simulink model "s_c_nbe_m32k"  (R2018a)
settings: Solver=VariableStepDiscrete  StartTime=0.0  StopTime=1000  RelTol=1e-3
undefined symbols (not defined in the file): fft_stages, n_taps, output_bits, pfb_coeff_gen_calc, xengbits
libraries: xbsIndex_r4 x23714, casper_library_misc x17, xps_library x4, casper_library_scopes x4, xbsReplacements_r4 x4
(part 18 of 171)

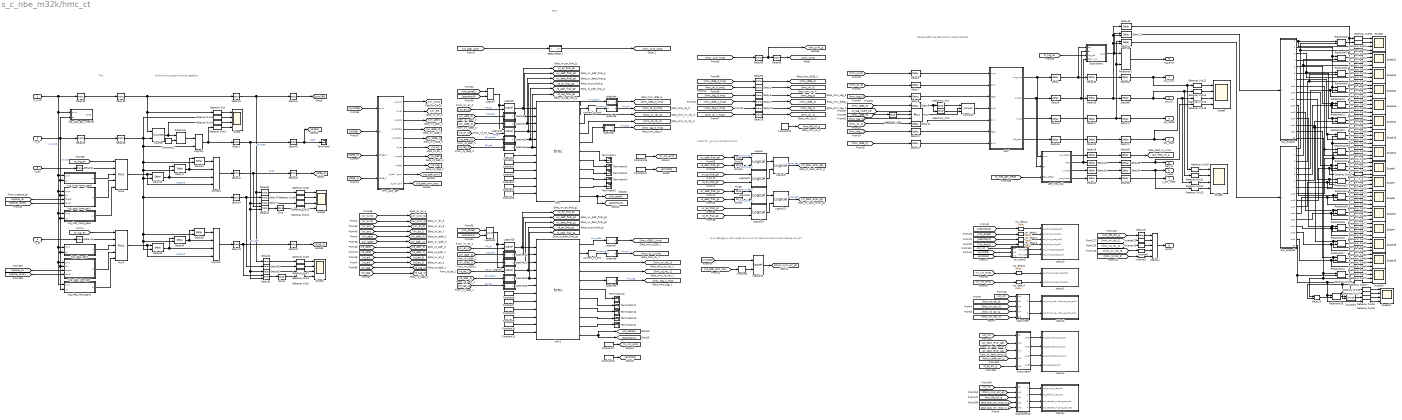
== system s_c_nbe_m32k/hmc_ct ==
  note: Double buffer the data to form output packets
  note: TVG
  note: Write two successive words together.
  note: Sync debugging - did we get two syncs
      | so close we weren't even reading out yet?
  note: Check for _en sync and bank errors
  note: HMC
  in_sync : Inport
  in_dv : Inport  Port=2
  in_d0 : Inport  Port=3
  in_d1 : Inport  Port=4
  Concat13 : xbsIndex_r4/Concat  num_inputs=3  dbl_ovrd=off  block_type=concat
  Concat2 : xbsIndex_r4/Concat  num_inputs=4  dbl_ovrd=off  block_type=concat
  Concat3 : xbsIndex_r4/Concat  num_inputs=4  dbl_ovrd=off  block_type=concat
  Constant{,3,6,9} (4 alike) : xbsIndex_r4/Constant  const=0  gui_display_data_type=Boolean  arith_type=Boolean  n_bits=16  bin_pt=14  preci_type=Single  exp_width=8  frac_width=24  explicit_period=on  period=1  equ=P=C  opselect=C  inp2=PCIN>>17  opr=+  inp1=P  carry=CIN  dbl_ovrd=off  block_type=constant
  Constant{1,4,7,10} (4 alike) : xbsIndex_r4/Constant  const=0  gui_display_data_type=Fixed-point  arith_type=Unsigned  n_bits=27  bin_pt=0  preci_type=Single  exp_width=8  frac_width=24  explicit_period=on  period=1  equ=P=C  opselect=C  inp2=PCIN>>17  opr=+  inp1=P  carry=CIN  dbl_ovrd=off  block_type=constant
  Constant11 : xbsIndex_r4/Constant  const=0  gui_display_data_type=Fixed-point  arith_type=Unsigned  n_bits=9  bin_pt=0  preci_type=Single  exp_width=8  frac_width=24  explicit_period=on  period=1  equ=P=C  opselect=C  inp2=PCIN>>17  opr=+  inp1=P  carry=CIN  dbl_ovrd=off  block_type=constant
  Constant12 : xbsIndex_r4/Constant  const=3  gui_display_data_type=Fixed-point  arith_type=Unsigned  n_bits=2  bin_pt=0  preci_type=Single  exp_width=8  frac_width=24  explicit_period=on  period=1  equ=P=C  opselect=C  inp2=PCIN>>17  opr=+  inp1=P  carry=CIN  dbl_ovrd=off  block_type=constant
  Constant13 : xbsIndex_r4/Constant  const=0  gui_display_data_type=Boolean  arith_type=Boolean  n_bits=1  bin_pt=0  preci_type=Single  exp_width=8  frac_width=24  explicit_period=on  period=1  equ=P=C  opselect=C  inp2=PCIN>>17  opr=+  inp1=P  carry=CIN  dbl_ovrd=off  block_type=constant
  Constant14 : xbsIndex_r4/Constant  const=0  gui_display_data_type=Fixed-point  arith_type=Unsigned  n_bits=7  bin_pt=0  preci_type=Single  exp_width=8  frac_width=24  explicit_period=on  period=1  equ=P=C  opselect=C  inp2=PCIN>>17  opr=+  inp1=P  carry=CIN  dbl_ovrd=off  block_type=constant
  Constant15 : xbsIndex_r4/Constant  const=0  gui_display_data_type=Fixed-point  arith_type=Unsigned  n_bits=16  bin_pt=0  preci_type=Single  exp_width=8  frac_width=24  explicit_period=on  period=1  equ=P=C  opselect=C  inp2=PCIN>>17  opr=+  inp1=P  carry=CIN  dbl_ovrd=off  block_type=constant
  Constant16 : xbsIndex_r4/Constant  const=0  gui_display_data_type=Fixed-point  arith_type=Unsigned  n_bits=7  bin_pt=0  preci_type=Single  exp_width=8  frac_width=24  explicit_period=on  period=1  equ=P=C  opselect=C  inp2=PCIN>>17  opr=+  inp1=P  carry=CIN  dbl_ovrd=off  block_type=constant
  Constant17 : xbsIndex_r4/Constant  const=0  gui_display_data_type=Fixed-point  arith_type=Unsigned  n_bits=16  bin_pt=0  preci_type=Single  exp_width=8  frac_width=24  explicit_period=on  period=1  equ=P=C  opselect=C  inp2=PCIN>>17  opr=+  inp1=P  carry=CIN  dbl_ovrd=off  block_type=constant
  Constant2 : xbsIndex_r4/Constant  const=0  gui_display_data_type=Fixed-point  arith_type=Unsigned  n_bits=256  bin_pt=0  preci_type=Single  exp_width=8  frac_width=24  explicit_period=on  period=1  equ=P=C  opselect=C  inp2=PCIN>>17  opr=+  inp1=P  carry=CIN  dbl_ovrd=off  block_type=constant
  Constant5 : xbsIndex_r4/Constant  const=0  gui_display_data_type=Fixed-point  arith_type=Unsigned  n_bits=9  bin_pt=0  preci_type=Single  exp_width=8  frac_width=24  explicit_period=on  period=1  equ=P=C  opselect=C  inp2=PCIN>>17  opr=+  inp1=P  carry=CIN  dbl_ovrd=off  block_type=constant
  Constant8 : xbsIndex_r4/Constant  const=0  gui_display_data_type=Fixed-point  arith_type=Unsigned  n_bits=256  bin_pt=0  preci_type=Single  exp_width=8  frac_width=24  explicit_period=on  period=1  equ=P=C  opselect=C  inp2=PCIN>>17  opr=+  inp1=P  carry=CIN  dbl_ovrd=off  block_type=constant
  Counter : xbsIndex_r4/Counter  cnt_type=Free Running  cnt_to=Inf  operation=Up  start_count=0  cnt_by_val=1  arith_type=Unsigned  n_bits=2  bin_pt=0  load_pin=off  rst=on  en=on  explicit_period=on  period=1  use_behavioral_HDL=off  implementation=Fabric  dbl_ovrd=off  block_type=counter
  Counter1 : xbsIndex_r4/Counter  cnt_type=Free Running  cnt_to=Inf  operation=Up  start_count=0  cnt_by_val=1  arith_type=Unsigned  n_bits=8  bin_pt=0  load_pin=off  rst=on  en=on  explicit_period=on  period=1  use_behavioral_HDL=off  implementation=Fabric  dbl_ovrd=off  block_type=counter
  Delay{,6,10,16} (4 alike) : xbsIndex_r4/Delay  rst=off  infoeditControl=Selection of Reset will increase slice count due to use of real FFs and instead of SRLs  en=off  latency=21  reg_retiming=on  dbl_ovrd=off  block_type=delay
      settings: infoedit=Hardware notes: A delay line is a chain, each link of which is an SRL16 or SRL32 followed by a flip-flop.
  Delay{1,5,7..9,11..13,15,25..29,35,39..40,42,54,61..62,78,93} (23 alike) : xbsIndex_r4/Delay  rst=off  infoeditControl=Selection of Reset will increase slice count due to use of real FFs and instead of SRLs  en=off  latency=2  reg_retiming=on  dbl_ovrd=off  block_type=delay
      settings: infoedit=Hardware notes: A delay line is a chain, each link of which is an SRL16 or SRL32 followed by a flip-flop.
  Delay{14,21..23,81} (5 alike) : xbsIndex_r4/Delay  rst=off  infoeditControl=Selection of Reset will increase slice count due to use of real FFs and instead of SRLs  en=on  latency=1  reg_retiming=off  dbl_ovrd=off  block_type=delay
      settings: infoedit=Hardware notes: A delay line is a chain, each link of which is an SRL16 or SRL32 followed by a flip-flop.
  Delay{2..4,17..19,43..45,63,66,72..73,75,85..86,89..90,94..95} (20 alike) : xbsIndex_r4/Delay  rst=off  infoeditControl=Selection of Reset will increase slice count due to use of real FFs and instead of SRLs  en=off  latency=1  reg_retiming=on  dbl_ovrd=off  block_type=delay
      settings: infoedit=Hardware notes: A delay line is a chain, each link of which is an SRL16 or SRL32 followed by a flip-flop.
  Delay{33..34,36,41} (4 alike) : xbsIndex_r4/Delay  rst=off  infoeditControl=Selection of Reset will increase slice count due to use of real FFs and instead of SRLs  en=off  latency=4  reg_retiming=on  dbl_ovrd=off  block_type=delay
      settings: infoedit=Hardware notes: A delay line is a chain, each link of which is an SRL16 or SRL32 followed by a flip-flop.
  Delay{46..47,51,60,64..65} (6 alike) : xbsIndex_r4/Delay  rst=off  infoeditControl=Selection of Reset will increase slice count due to use of real FFs and instead of SRLs  en=on  latency=1  reg_retiming=on  dbl_ovrd=off  block_type=delay
      settings: infoedit=Hardware notes: A delay line is a chain, each link of which is an SRL16 or SRL32 followed by a flip-flop.
  Delay{48,77,79..80,82..84} (7 alike) : xbsIndex_r4/Delay  rst=off  infoeditControl=Selection of Reset will increase slice count due to use of real FFs and instead of SRLs  en=off  latency=1  reg_retiming=off  dbl_ovrd=off  block_type=delay
      settings: infoedit=Hardware notes: A delay line is a chain, each link of which is an SRL16 or SRL32 followed by a flip-flop.
  Gateway Out{,1..87} (88 alike) : xbsIndex_r4/Gateway Out  inherit_from_input=off  hdl_port=off  rows=1  columns=1  UseAsDAC=off  DACChannel='1'  interface=None  automatic_assignment=on  address_offset=hex2dec('00')  intf_name=''  intf_description=''  timing_constraint=None  locs_specified=off  LOCs={}  io_standard={}  block_type=gatewayout
  Inverter{1..2,22..23} (4 alike) : xbsIndex_r4/Inverter  en=off  latency=1  dbl_ovrd=off  block_type=inv
  Inverter6 : xbsIndex_r4/Inverter  en=off  latency=0  dbl_ovrd=off  block_type=inv
  Logical{,1,8,19,21} (5 alike) : xbsIndex_r4/Logical  logical_function=AND  inputs=2  en=off  latency=0  precision=Full  arith_type=Unsigned  n_bits=16  bin_pt=0  align_bp=on  dbl_ovrd=off  block_type=logical
  Logical10 : xbsIndex_r4/Logical  logical_function=OR  inputs=2  en=off  latency=0  precision=Full  arith_type=Unsigned  n_bits=16  bin_pt=0  align_bp=on  dbl_ovrd=off  block_type=logical
  Logical{2,5,11,15,18} (5 alike) : xbsIndex_r4/Logical  logical_function=AND  inputs=2  en=off  latency=2  precision=Full  arith_type=Unsigned  n_bits=16  bin_pt=0  align_bp=on  dbl_ovrd=off  block_type=logical
  Logical20 : xbsIndex_r4/Logical  logical_function=OR  inputs=2  en=off  latency=0  precision=Full  arith_type=Unsigned  n_bits=16  bin_pt=0  align_bp=on  dbl_ovrd=off  block_type=logical
  Logical28 : xbsIndex_r4/Logical  logical_function=AND  inputs=2  en=off  latency=1  precision=Full  arith_type=Unsigned  n_bits=16  bin_pt=0  align_bp=on  dbl_ovrd=off  block_type=logical
  Logical4 : xbsIndex_r4/Logical  logical_function=OR  inputs=5  en=off  latency=1  precision=Full  arith_type=Unsigned  n_bits=16  bin_pt=0  align_bp=on  dbl_ovrd=off  block_type=logical
  Logical7 : xbsIndex_r4/Logical  logical_function=AND  inputs=2  en=off  latency=1  precision=Full  arith_type=Unsigned  n_bits=16  bin_pt=0  align_bp=on  dbl_ovrd=off  block_type=logical
  Mux : xbsIndex_r4/Mux  inputs=2  en=off  latency=2  precision=Full  arith_type=Unsigned  n_bits=16  bin_pt=14  quantization=Truncate  overflow=Wrap  dbl_ovrd=off  block_type=mux
  Mux3 : xbsIndex_r4/Mux  inputs=4  en=off  latency=2  precision=Full  arith_type=Unsigned  n_bits=16  bin_pt=14  quantization=Truncate  overflow=Wrap  dbl_ovrd=off  block_type=mux
  Mux4 : xbsIndex_r4/Mux  inputs=4  en=off  latency=2  precision=Full  arith_type=Unsigned  n_bits=16  bin_pt=14  quantization=Truncate  overflow=Wrap  dbl_ovrd=off  block_type=mux
  Relational : xbsIndex_r4/Relational  mode=a=b  op_type=Bool  en=off  latency=0  dbl_ovrd=off  block_type=relational
  Relational1 : xbsIndex_r4/Relational  mode=a!=b  op_type=Bool  en=off  latency=1  dbl_ovrd=off  block_type=relational
  Relational{2..18} (17 alike) : xbsIndex_r4/Relational  mode=a!=b  op_type=Bool  en=off  latency=0  dbl_ovrd=off  block_type=relational
  Scope{,1..21} (22 alike) : Scope  NumInputPorts=4
  Slice : xbsIndex_r4/Slice  nbits=16  boolean_output=off  mode=Upper Bit Location + Width  bit1=0  base1=MSB of Input  bit0=0  base0=LSB of Input  dbl_ovrd=off  block_type=slice
  Slice1 : xbsIndex_r4/Slice  nbits=16  boolean_output=off  mode=Upper Bit Location + Width  bit1=0  base1=MSB of Input  bit0=0  base0=LSB of Input  dbl_ovrd=off  block_type=slice
  Slice{8..9,12..13} (4 alike) : xbsIndex_r4/Slice  nbits=1  boolean_output=on  mode=Lower Bit Location + Width  bit1=0  base1=MSB of Input  bit0=input_len_bits - 2 + output_len_bits  base0=LSB of Input  dbl_ovrd=off  block_type=slice
  Subsystem : Subsystem
  Subsystem1 : Subsystem
  Subsystem22 : Subsystem  mask{n_bits_count=8}
      mask prompts: n_bits_count "Counter bits"
  Subsystem9 : Subsystem  mask{n_bits_count=8}
      mask prompts: n_bits_count "Counter bits"
  Terminator{,1..5,10..14} (11 alike) : Terminator
  bus_expand : Subsystem  mask(bus_expand){mode=divisions of equal size, outputNum=16, outputWidth=16, outputBinaryPt=0, outputArithmeticType=0, show_format=off, outputToWorkspace=off, variablePrefix=out, outputToModelAsWell=on}
      mask prompts: outputNum "Number of outputs:"; outputWidth "Output width:"; outputBinaryPt "Output binary point position:"; outputArithmeticType "Output arithmetic type (ufix=0, fix=1, bool=2):"; show_format "Print format string?"; outputToWorkspace "Output to workspace?"; variablePrefix "Variable name prefix:"; outputToModelAsWell "Output to model as well?"
      mask help:
      | Expands a 'bus' made using a bus_create or Xilinx
      | concat block.
      | The input will be divided into the specified number
      | of outputs with the specified arithmetic types.
      | Divisions are made from most significant bit.
      mask init: same as s_c_nbe_m32k/bus_expand1
      settings: AttributesFormatString=16 outputs
      mask TypeOptions mode: divisions of equal size | divisions of arbitrary size
      mask Callback mode: bus_expand_callback();
      mask Callback outputWidth: bus_expand_callback();
      mask Callback outputToWorkspace: bus_expand_callback();
  bus_expand1 : Subsystem  mask(bus_expand){mode=divisions of equal size, outputNum=16, outputWidth=16, outputBinaryPt=0, outputArithmeticType=0, show_format=off, outputToWorkspace=off, variablePrefix=out, outputToModelAsWell=on}
      mask prompts: outputNum "Number of outputs:"; outputWidth "Output width:"; outputBinaryPt "Output binary point position:"; outputArithmeticType "Output arithmetic type (ufix=0, fix=1, bool=2):"; show_format "Print format string?"; outputToWorkspace "Output to workspace?"; variablePrefix "Variable name prefix:"; outputToModelAsWell "Output to model as well?"
      mask help:
      | Expands a 'bus' made using a bus_create or Xilinx
      | concat block.
      | The input will be divided into the specified number
      | of outputs with the specified arithmetic types.
      | Divisions are made from most significant bit.
      mask init: same as s_c_nbe_m32k/bus_expand1
      settings: AttributesFormatString=16 outputs
      mask TypeOptions mode: divisions of equal size | divisions of arbitrary size
      mask Callback mode: bus_expand_callback();
      mask Callback outputWidth: bus_expand_callback();
      mask Callback outputToWorkspace: bus_expand_callback();
  convert_rd_en1 : xbsIndex_r4/Convert  gui_display_data_type=Boolean  arith_type=Boolean  n_bits=128  bin_pt=0  float_type=Single  exp_bits=8  fraction_bits=24  quantization=Truncate  overflow=Wrap  en=off  latency=0  pipeline=off  dbl_ovrd=off  block_type=convert
      settings: xl_area=[0, 0, 0, 0, 0, 0, 0]
  convert_rd_en4 : xbsIndex_r4/Convert  gui_display_data_type=Boolean  arith_type=Boolean  n_bits=128  bin_pt=0  float_type=Single  exp_bits=8  fraction_bits=24  quantization=Truncate  overflow=Wrap  en=off  latency=0  pipeline=off  dbl_ovrd=off  block_type=convert
      settings: xl_area=[0, 0, 0, 0, 0, 0, 0]
  edge_detect1 : Subsystem  mask(edge_detect){edge=Rising, polarity=Active High, x_in=[0 0.08 0.08 0.16 0.16 0.24 0.24 0.32 0.32 0.4], y_in=[-1 -1  1  1  1  1  1  1  1  1], x_out=[0.6 0.68 0.68 0.76 0.76 0.84 0.84 0.92 0.92 1], y_out=[-1 -1  1  1 -1 -1 -1 -1 -1 -1]}
      mask prompts: edge "Edge Type"; polarity "Output Polarity"; x_in "Input X Positions"; y_in "Input Y Positions"; x_out "Output X Positions"; y_out "Output Y Positions"
      mask help: Output is active for one-cycle after each edge of the specified type (i.e. rising, falling or both).
      mask init: same as s_c_nbe_m32k/edge_detect1
      settings: AttributesFormatString=|
      | rising edges
      | active high
      mask Help: Output is active for one-cycle after each edge of the specified type (i.e. rising, falling, or both).  Latency is zero.
      mask TypeOptions edge: Rising | Falling | Both
      mask TypeOptions polarity: Active High | Active Low
      mask Display:
      | plot(x_in_num,0.5+y_in_num*0.2);
      | plot(x_out_num,0.5+y_out_num*0.2);
  err_latch3 : Subsystem
  gen_freq_calc : Subsystem  mask{pkt_len_bits=5, lat=3}
      mask prompts: pkt_len_bits "Packet length bits"; lat "Latency"
      mask init:
      | display_string = sprintf('latency=%i', 7 * lat);
      | set_param(gcb, 'AttributesFormatString', display_string);
      settings: AttributesFormatString=latency=21
  hmc : xps_library/Memory/hmc  Tag=xps:hmc  mez=1  sim_depth=(input_len_bits-1) + output_len_bits + 1  sim_latency=5  sim_rand=on
      settings: SourceProductName=CASPER XPS Blockset
  hmc1 : xps_library/Memory/hmc  Tag=xps:hmc  mez=2  sim_depth=(input_len_bits-1) + output_len_bits + 1  sim_latency=5  sim_rand=on
      settings: SourceProductName=CASPER XPS Blockset
  hmc_addr_gen : Subsystem  mask{invec_bits=input_len_bits-2, outvec_bits=output_len_bits, max_x_boards_bits=max_x_boards_bits, max_x_per_board_bits=max_x_per_board_bits, n_bits_chans_per_word=4}
      mask prompts: invec_bits "Input vector bits"; outvec_bits "Output vector bits"; max_x_boards_bits "Max number x boards (2^?)"; max_x_per_board_bits "max xengines per board (2^?)"; n_bits_chans_per_word "channels per input word (2^?)"
      mask init:
      | vec_len = 2^invec_bits * 2^outvec_bits;
      | mystr = sprintf('2^%i x 2^%i = %i', invec_bits, outvec_bits, vec_len);
      | set_param(gcb, 'AttributesFormatString', mystr);
      settings: AttributesFormatString=2^11 x 2^8 = 524288
  obuf : Subsystem  mask{output_vec_bits=output_len_bits, pkt_buffer_latency=4, omux_latency=3}
      mask prompts: output_vec_bits "CT output vector bits"; pkt_buffer_latency "Output buffer latency"; omux_latency "Output mux latency"
  pipeline : Subsystem  Tag=cmac_delinked  mask(pipeline){csp_latency=2}
      mask prompts: csp_latency "Latency"
      mask help:
      | An explicitly laid-out delay line to avoid mapping to SRL16s
      | for use in pipelining to help achieve timing closure.
      mask init:
      | pipeline_init(gcb,'latency',csp_latency);
      settings: AttributesFormatString=Latency = %<latency>
      mask Display:
      | port_label('input', 1, 'd');
      | port_label('output', 1, 'q');
      | disp(['Z^-', num2str(csp_latency)]);
  pipeline1 : Subsystem  Tag=cmac_delinked  mask(pipeline){csp_latency=2}
      mask prompts: csp_latency "Latency"
      mask help:
      | An explicitly laid-out delay line to avoid mapping to SRL16s
      | for use in pipelining to help achieve timing closure.
      mask init:
      | pipeline_init(gcb,'latency',csp_latency);
      settings: AttributesFormatString=Latency = %<latency>
      mask Display:
      | port_label('input', 1, 'd');
      | port_label('output', 1, 'q');
      | disp(['Z^-', num2str(csp_latency)]);
  pipeline10 : Subsystem  Tag=cmac_delinked  mask(pipeline){csp_latency=2}
      mask prompts: csp_latency "Latency"
      mask help:
      | An explicitly laid-out delay line to avoid mapping to SRL16s
      | for use in pipelining to help achieve timing closure.
      mask init:
      | pipeline_init(gcb,'latency',csp_latency);
      settings: AttributesFormatString=Latency = %<latency>
      mask Display:
      | port_label('input', 1, 'd');
      | port_label('output', 1, 'q');
      | disp(['Z^-', num2str(csp_latency)]);
  pipeline11 : Subsystem  Tag=cmac_delinked  mask(pipeline){csp_latency=2}
      mask prompts: csp_latency "Latency"
      mask help:
      | An explicitly laid-out delay line to avoid mapping to SRL16s
      | for use in pipelining to help achieve timing closure.
      mask init:
      | pipeline_init(gcb,'latency',csp_latency);
      settings: AttributesFormatString=Latency = %<latency>
      mask Display:
      | port_label('input', 1, 'd');
      | port_label('output', 1, 'q');
      | disp(['Z^-', num2str(csp_latency)]);
  pipeline12 : Subsystem  Tag=cmac_delinked  mask(pipeline){csp_latency=2}
      mask prompts: csp_latency "Latency"
      mask help:
      | An explicitly laid-out delay line to avoid mapping to SRL16s
      | for use in pipelining to help achieve timing closure.
      mask init:
      | pipeline_init(gcb,'latency',csp_latency);
      settings: AttributesFormatString=Latency = %<latency>
      mask Display:
      | port_label('input', 1, 'd');
      | port_label('output', 1, 'q');
      | disp(['Z^-', num2str(csp_latency)]);
  pipeline13 : Subsystem  Tag=cmac_delinked  mask(pipeline){csp_latency=2}
      mask prompts: csp_latency "Latency"
      mask help:
      | An explicitly laid-out delay line to avoid mapping to SRL16s
      | for use in pipelining to help achieve timing closure.
      mask init:
      | pipeline_init(gcb,'latency',csp_latency);
      settings: AttributesFormatString=Latency = %<latency>
      mask Display:
      | port_label('input', 1, 'd');
      | port_label('output', 1, 'q');
      | disp(['Z^-', num2str(csp_latency)]);
  pipeline2 : Subsystem  Tag=cmac_delinked  mask(pipeline){csp_latency=2}
      mask prompts: csp_latency "Latency"
      mask help:
      | An explicitly laid-out delay line to avoid mapping to SRL16s
      | for use in pipelining to help achieve timing closure.
      mask init:
      | pipeline_init(gcb,'latency',csp_latency);
      settings: AttributesFormatString=Latency = %<latency>
      mask Display:
      | port_label('input', 1, 'd');
      | port_label('output', 1, 'q');
      | disp(['Z^-', num2str(csp_latency)]);
  pipeline3 : Subsystem  Tag=cmac_delinked  mask(pipeline){csp_latency=2}
      mask prompts: csp_latency "Latency"
      mask help:
      | An explicitly laid-out delay line to avoid mapping to SRL16s
      | for use in pipelining to help achieve timing closure.
      mask init:
      | pipeline_init(gcb,'latency',csp_latency);
      settings: AttributesFormatString=Latency = %<latency>
      mask Display:
      | port_label('input', 1, 'd');
      | port_label('output', 1, 'q');
      | disp(['Z^-', num2str(csp_latency)]);
  pipeline4 : Subsystem  Tag=cmac_delinked  mask(pipeline){csp_latency=2}
      mask prompts: csp_latency "Latency"
      mask help:
      | An explicitly laid-out delay line to avoid mapping to SRL16s
      | for use in pipelining to help achieve timing closure.
      mask init:
      | pipeline_init(gcb,'latency',csp_latency);
      settings: AttributesFormatString=Latency = %<latency>
      mask Display:
      | port_label('input', 1, 'd');
      | port_label('output', 1, 'q');
      | disp(['Z^-', num2str(csp_latency)]);
  pipeline5 : Subsystem  Tag=cmac_delinked  mask(pipeline){csp_latency=2}
      mask prompts: csp_latency "Latency"
      mask help:
      | An explicitly laid-out delay line to avoid mapping to SRL16s
      | for use in pipelining to help achieve timing closure.
      mask init:
      | pipeline_init(gcb,'latency',csp_latency);
      settings: AttributesFormatString=Latency = %<latency>
      mask Display:
      | port_label('input', 1, 'd');
      | port_label('output', 1, 'q');
      | disp(['Z^-', num2str(csp_latency)]);
  pipeline6 : Subsystem  Tag=cmac_delinked  mask(pipeline){csp_latency=2}
      mask prompts: csp_latency "Latency"
      mask help:
      | An explicitly laid-out delay line to avoid mapping to SRL16s
      | for use in pipelining to help achieve timing closure.
      mask init:
      | pipeline_init(gcb,'latency',csp_latency);
      settings: AttributesFormatString=Latency = %<latency>
      mask Display:
      | port_label('input', 1, 'd');
      | port_label('output', 1, 'q');
      | disp(['Z^-', num2str(csp_latency)]);
  pipeline7 : Subsystem  Tag=cmac_delinked  mask(pipeline){csp_latency=2}
      mask prompts: csp_latency "Latency"
      mask help:
      | An explicitly laid-out delay line to avoid mapping to SRL16s
      | for use in pipelining to help achieve timing closure.
      mask init:
      | pipeline_init(gcb,'latency',csp_latency);
      settings: AttributesFormatString=Latency = %<latency>
      mask Display:
      | port_label('input', 1, 'd');
      | port_label('output', 1, 'q');
      | disp(['Z^-', num2str(csp_latency)]);
  pipeline8 : Subsystem  Tag=cmac_delinked  mask(pipeline){csp_latency=2}
      mask prompts: csp_latency "Latency"
      mask help:
      | An explicitly laid-out delay line to avoid mapping to SRL16s
      | for use in pipelining to help achieve timing closure.
      mask init:
      | pipeline_init(gcb,'latency',csp_latency);
      settings: AttributesFormatString=Latency = %<latency>
      mask Display:
      | port_label('input', 1, 'd');
      | port_label('output', 1, 'q');
      | disp(['Z^-', num2str(csp_latency)]);
  pipeline9 : Subsystem  Tag=cmac_delinked  mask(pipeline){csp_latency=2}
      mask prompts: csp_latency "Latency"
      mask help:
      | An explicitly laid-out delay line to avoid mapping to SRL16s
      | for use in pipelining to help achieve timing closure.
      mask init:
      | pipeline_init(gcb,'latency',csp_latency);
      settings: AttributesFormatString=Latency = %<latency>
      mask Display:
      | port_label('input', 1, 'd');
      | port_label('output', 1, 'q');
      | disp(['Z^-', num2str(csp_latency)]);
  rst_delay{1..5,7} (6 alike) : xbsIndex_r4/Delay  rst=off  infoeditControl=Selection of Reset will increase slice count due to use of real FFs and instead of SRLs  en=off  latency=1  reg_retiming=on  dbl_ovrd=off  block_type=delay
      settings: infoedit=Hardware notes: A delay line is a chain, each link of which is an SRL16 or SRL32 followed by a flip-flop.
  spectrum_ctr2 : xbsIndex_r4/Slice  nbits=256 - (32 + 10)  boolean_output=off  mode=Lower Bit Location + Width  bit1=-1  base1=MSB of Input  bit0=32 + 10  base0=LSB of Input  dbl_ovrd=off  block_type=slice
  spectrum_ctr3 : xbsIndex_r4/Slice  nbits=32  boolean_output=off  mode=Lower Bit Location + Width  bit1=-1  base1=MSB of Input  bit0=0  base0=LSB of Input  dbl_ovrd=off  block_type=slice
  spectrum_ctr4 : xbsIndex_r4/Slice  nbits=10  boolean_output=off  mode=Lower Bit Location + Width  bit1=-1  base1=MSB of Input  bit0=32  base0=LSB of Input  dbl_ovrd=off  block_type=slice
  status0 : Subsystem  Tag=xps:sw_reg  AncestorBlock=xps_library/Memory/software_register  mask(swreg){io_dir=To Processor, io_delay=0, init_val=0, sample_period=1, names=[hmc_post_pol0 hmc_init_pol0 hmc_post_pol1 hmc_init_pol1 hmc_errstat_pol0 hmc_errstat_pol1], bitwidths=[1 1 1 1 7 7], bin_pts=0, arith_types=[2 2 2 2 0 0], sim_port=off, show_format=on}
      mask prompts: io_dir "I/O direction"; io_delay "I/O delay"; init_val "Initial Value"; sample_period "Sample period"; names "Bitfield names [msb...lsb]"; bitwidths "Bitfield widths"; bin_pts "Bitfield binary pts"; arith_types "Bitfield types, ufix=0, fix=1, bool=2"; sim_port "Provide sim input/output?"; show_format "Print format string?"
      mask help: A 32-bit software-accessible register. Can be divided into bitfields of varying widths and types using the fields in the block mask.
      mask init:
      | swreg_init(gcb)
      settings: AttributesFormatString=6 outputs:b,b,b,b,uf7.0,uf7.0 = 18 bits
      mask TypeOptions io_dir: To Processor | From Processor
      mask Callback io_dir:
      | mask_enables = get_param(gcb, 'MaskEnables');
      | mask_names = get_param(gcb, 'MaskNames');
      | if strcmp(get_param(gcb, 'io_dir'), 'To Processor'),
      |     mask_enables{ismember(mask_names, 'sample_period')} = 'off';
      | else
      |     mask_enables{ismember(mask_names, 'sample_period')} = 'on';
      | end
      | set_param(gcb, 'MaskEnables', mask_enables);
      mask DialogControl ParameterTabVar0 Prompt: Setup
  status1 : Subsystem  Tag=xps:sw_reg  AncestorBlock=xps_library/Memory/software_register  mask(swreg){io_dir=To Processor, io_delay=0, init_val=0, sample_period=1, names=[hmc_crc_err_cnt_pol0 hmc_crc_err_cnt_pol1], bitwidths=16, bin_pts=0, arith_types=0, sim_port=off, show_format=on}
      mask prompts: io_dir "I/O direction"; io_delay "I/O delay"; init_val "Initial Value"; sample_period "Sample period"; names "Bitfield names [msb...lsb]"; bitwidths "Bitfield widths"; bin_pts "Bitfield binary pts"; arith_types "Bitfield types, ufix=0, fix=1, bool=2"; sim_port "Provide sim input/output?"; show_format "Print format string?"
      mask help: A 32-bit software-accessible register. Can be divided into bitfields of varying widths and types using the fields in the block mask.
      mask init:
      | swreg_init(gcb)
      settings: AttributesFormatString=2 outputs:uf16.0,uf16.0 = 32 bits
      mask TypeOptions io_dir: To Processor | From Processor
      mask Callback io_dir:
      | mask_enables = get_param(gcb, 'MaskEnables');
      | mask_names = get_param(gcb, 'MaskNames');
      | if strcmp(get_param(gcb, 'io_dir'), 'To Processor'),
      |     mask_enables{ismember(mask_names, 'sample_period')} = 'off';
      | else
      |     mask_enables{ismember(mask_names, 'sample_period')} = 'on';
      | end
      | set_param(gcb, 'MaskEnables', mask_enables);
      mask DialogControl ParameterTabVar0 Prompt: Setup
  status2 : Subsystem  Tag=xps:sw_reg  AncestorBlock=xps_library/Memory/software_register  mask(swreg){io_dir=To Processor, io_delay=0, init_val=0, sample_period=1, names=[hmc_overflow_err_cnt_pol0 hmc_overflow_err_cnt_pol1], bitwidths=16, bin_pts=0, arith_types=0, sim_port=off, show_format=on}
      mask prompts: io_dir "I/O direction"; io_delay "I/O delay"; init_val "Initial Value"; sample_period "Sample period"; names "Bitfield names [msb...lsb]"; bitwidths "Bitfield widths"; bin_pts "Bitfield binary pts"; arith_types "Bitfield types, ufix=0, fix=1, bool=2"; sim_port "Provide sim input/output?"; show_format "Print format string?"
      mask help: A 32-bit software-accessible register. Can be divided into bitfields of varying widths and types using the fields in the block mask.
      mask init:
      | swreg_init(gcb)
      settings: AttributesFormatString=2 outputs:uf16.0,uf16.0 = 32 bits
      mask TypeOptions io_dir: To Processor | From Processor
      mask Callback io_dir:
      | mask_enables = get_param(gcb, 'MaskEnables');
      | mask_names = get_param(gcb, 'MaskNames');
      | if strcmp(get_param(gcb, 'io_dir'), 'To Processor'),
      |     mask_enables{ismember(mask_names, 'sample_period')} = 'off';
      | else
      |     mask_enables{ismember(mask_names, 'sample_period')} = 'on';
      | end
      | set_param(gcb, 'MaskEnables', mask_enables);
      mask DialogControl ParameterTabVar0 Prompt: Setup
  status3 : Subsystem  Tag=xps:sw_reg  AncestorBlock=xps_library/Memory/software_register  mask(swreg){io_dir=To Processor, io_delay=0, init_val=0, sample_period=1, names=[bank_err_cnt_pol0 bank_err_cnt_pol1 obuff_bank_err_cnt rd_go_err_cnt], bitwidths=8, bin_pts=0, arith_types=0, sim_port=off, show_format=on}
      mask prompts: io_dir "I/O direction"; io_delay "I/O delay"; init_val "Initial Value"; sample_period "Sample period"; names "Bitfield names [msb...lsb]"; bitwidths "Bitfield widths"; bin_pts "Bitfield binary pts"; arith_types "Bitfield types, ufix=0, fix=1, bool=2"; sim_port "Provide sim input/output?"; show_format "Print format string?"
      mask help: A 32-bit software-accessible register. Can be divided into bitfields of varying widths and types using the fields in the block mask.
      mask init:
      | swreg_init(gcb)
      settings: AttributesFormatString=4 outputs:uf8.0,uf8.0,uf8.0,uf8.0 = 32 bits
      mask TypeOptions io_dir: To Processor | From Processor
      mask Callback io_dir:
      | mask_enables = get_param(gcb, 'MaskEnables');
      | mask_names = get_param(gcb, 'MaskNames');
      | if strcmp(get_param(gcb, 'io_dir'), 'To Processor'),
      |     mask_enables{ismember(mask_names, 'sample_period')} = 'off';
      | else
      |     mask_enables{ismember(mask_names, 'sample_period')} = 'on';
      | end
      | set_param(gcb, 'MaskEnables', mask_enables);
      mask DialogControl ParameterTabVar0 Prompt: Setup
  status4 : Subsystem  Tag=xps:sw_reg  AncestorBlock=xps_library/Memory/software_register  mask(swreg){io_dir=To Processor, io_delay=0, init_val=0, sample_period=1, names=[sync_in_err_cnt fifo_full_err_cnt reorder_missing_err_cnt reorder_missing_err_cnt1], bitwidths=8, bin_pts=0, arith_types=0, sim_port=off, show_format=on}
      mask prompts: io_dir "I/O direction"; io_delay "I/O delay"; init_val "Initial Value"; sample_period "Sample period"; names "Bitfield names [msb...lsb]"; bitwidths "Bitfield widths"; bin_pts "Bitfield binary pts"; arith_types "Bitfield types, ufix=0, fix=1, bool=2"; sim_port "Provide sim input/output?"; show_format "Print format string?"
      mask help: A 32-bit software-accessible register. Can be divided into bitfields of varying widths and types using the fields in the block mask.
      mask init:
      | swreg_init(gcb)
      settings: AttributesFormatString=4 outputs:uf8.0,uf8.0,uf8.0,uf8.0 = 32 bits
      mask TypeOptions io_dir: To Processor | From Processor
      mask Callback io_dir:
      | mask_enables = get_param(gcb, 'MaskEnables');
      | mask_names = get_param(gcb, 'MaskNames');
      | if strcmp(get_param(gcb, 'io_dir'), 'To Processor'),
      |     mask_enables{ismember(mask_names, 'sample_period')} = 'off';
      | else
      |     mask_enables{ismember(mask_names, 'sample_period')} = 'on';
      | end
      | set_param(gcb, 'MaskEnables', mask_enables);
      mask DialogControl ParameterTabVar0 Prompt: Setup
  tvg_data_gen1 : Subsystem
  tvg_data_gen_oneshot : Subsystem
      mask Display:
      | color('red');
      | disp('ONE SHOT!!');
      | % color('green');
      | % port_label('input', 1, 'dv')
      | % color('red');
      | % port_label('output', 1, 'err')
  tvg_data_tone_gen : Subsystem
  tvg_data_tone_gen1 : Subsystem
  tvg_freq_ramp_gen0 : Subsystem
  tvg_freq_ramp_gen1 : Subsystem
  tvg_time_ramp_gen0 : Subsystem
  out_sync : Outport
  out_dv : Outport  Port=2
  out_d256 : Outport  Port=3
  pkt_start : Outport  Port=4
  freq_id : Outport  Port=5
  x_index : Outport  Port=6
  x_pkt_index : Outport  Port=7
  error0 : Outport  Port=8
  tvg_error : Outport  Port=9
  tag scope: cthmc_sync_err_g0=global, hmc_fifo_full_g=global, hmc_sync_g=global, raw_freq_ctr_g=global, rd_addr_final_g0=global, rd_addr_final_g1=global, rd_en_final_g0=global, rd_en_final_g1=global, rd_tag_final_g0=global, wr_addr_final_g0=global, wr_addr_final_g1=global, wr_data_final_g0=global, wr_data_final_g1=global, wr_en_final_g0=global, wr_en_final_g1=global
  wires:
  Delay6/1 -> Subsystem1/2(en), Delay26/1
  Delay10/1 -> Delay27/1
  Delay16/1 -> Delay28/1
  Delay9/1 -> spectrum_ctr2/1, spectrum_ctr3/1
  [hmc_sync] -> Delay5/1
  [hmc_dv_0] -> Delay7/1
  [hmc_tag_0] -> Delay8/1
  [ct_tag_insert_sel] -> Mux/1
  [hmc_d256_0] -> spectrum_ctr4/1
  spectrum_ctr4/1 -> Mux/2
  [hmc_tag_0] -> Mux/3
  Concat13/1 -> obuf/4(din0)
  spectrum_ctr3/1 -> Concat13/3
  Mux/1 -> Concat13/2
  spectrum_ctr2/1 -> Concat13/1
  Delay8/1 -> obuf/3(tag0)
  Delay7/1 -> obuf/2(dv0)
  Delay5/1 -> obuf/1(sync)
  obuf/4(pkt_start) -> Delay16/1
  obuf/3(out_d) -> Delay10/1
  obuf/2(out_dv) -> gen_freq_calc/2(dv), Delay6/1
  obuf/1(out_sync) -> gen_freq_calc/1(sync), Delay/1
  in_d0/1 -> Delay34/1
  [ct_tvg_en] -> Mux3/1
  Delay35/1 -> Delay15/1, Gateway Out/1, Counter/1
  Concat3/1 -> Delay42/1
  Mux3/1 -> Concat3/4, Delay46/1  "data128"
  in_dv/1 -> Delay33/1, tvg_data_gen_oneshot/2(dv), tvg_data_tone_gen1/2(dv), tvg_freq_ramp_gen1/2(dv), tvg_data_tone_gen/2(dv), tvg_data_gen1/2(dv), tvg_freq_ramp_gen0/2(dv), tvg_time_ramp_gen0/2(dv)  "dv128"
  in_sync/1 -> tvg_data_gen_oneshot/1(sync), tvg_data_tone_gen1/1(sync), tvg_freq_ramp_gen1/1(sync), tvg_data_tone_gen/1(sync), tvg_data_gen1/1(sync), tvg_freq_ramp_gen0/1(sync), tvg_time_ramp_gen0/1(sync), Delay36/1  "sync128"
  Delay33/1 -> Delay39/1
  Delay36/1 -> Delay35/1
  [rd_addr_arm_raw] -> Inverter6/1
  [sync256] -> Logical15/1
  Inverter6/1 -> Logical15/2
  Logical15/1 -> [cthmc_sync_err_g0]
  [tvgtone_p1] -> tvg_data_tone_gen/3(target)
  [tvgtone_level1] -> tvg_data_tone_gen/4(level)
  Delay15/1 -> Delay44/1, Delay84/1, Delay80/1  "sync256"
  Delay42/1 -> Delay43/1, Delay14/1  "d256"
  Delay1/1 -> Delay45/1, Delay77/1, Delay81/2, Delay82/1, Delay14/2  "dv_256"
  Delay45/1 -> [dv256], Terminator/1  "ORIG"
  Delay43/1 -> [d256_0]
  Delay44/1 -> [sync256]
  Delay34/1 -> Mux3/2
  [wr_addr] -> [wr_addr_0]
  [rd_addr] -> [rd_addr_1]
  [rd_tag] -> [rd_tag_0]
  [wr_sync] -> [wr_sync_1]
  [wr_addr_final_g0] -> Slice12/1
  [rd_addr_final_g0] -> Slice13/1
  Slice13/1 -> Logical/2  "final_rd_bank"
  Slice12/1 -> Logical/1  "final_wr_bank"
  Logical/1 -> Logical8/1
  Logical10/1 -> Logical8/2
  [wr_en_final_g0] -> Logical10/1
  [rd_en_final_g0] -> Logical10/2
  Logical8/1 -> [ct_bank_error_g0]  "same_bank"
  [wr_addr_final_g1] -> Slice8/1
  [rd_addr_final_g1] -> Slice9/1
  Slice9/1 -> Logical19/2  "final_rd_bank"
  Slice8/1 -> Logical19/1  "final_wr_bank"
  Logical19/1 -> Logical21/1
  Logical20/1 -> Logical21/2
  [wr_en_final_g1] -> Logical20/1
  [rd_en_final_g1] -> Logical20/2
  Logical21/1 -> [ct_bank_error_g1]  "same_bank"
  [sync256] -> hmc_addr_gen/1(sync)
  [d256_0] -> hmc_addr_gen/3(d256_0)
  hmc_addr_gen/1(wr_sync) -> [wr_sync]
  hmc_addr_gen/10(rd_arm_raw) -> [rd_addr_arm_raw]
  [hmc_sync_tmp] -> Delay89/1
  Delay89/1 -> Delay93/1, [hmc_sync_g]
  [hmc_d256_0_tmp] -> Delay90/1
  Delay90/1 -> [hmc_d256_0]
  [hmc_dv_0_tmp] -> Delay2/1
  Delay2/1 -> [hmc_dv_0]
  [hmc_tag_0_tmp] -> Delay3/1
  Delay3/1 -> [hmc_tag_0]
  Delay93/1 -> [hmc_sync]
  gen_freq_calc/1(raw_ctr64) -> Delay29/1
  gen_freq_calc/2(freq) -> Subsystem1/4(frequency), Delay40/1
  gen_freq_calc/3(x_index) -> Delay61/1
  gen_freq_calc/4(x_pkt_index) -> Delay62/1
  [ct_freq_gen_offset] -> gen_freq_calc/3(freq_offset)
  err_latch3/1(latched0) -> status0/5(out_hmc_errstat_pol0)
  err_latch3/2(latched1) -> status0/6(out_hmc_errstat_pol1)
  [errstat0] -> err_latch3/2(in0)
  [errstat1] -> err_latch3/3(in1)
  [cnt_rst] -> err_latch3/1(rst)
  [rx_crc_err0] -> rst_delay3/1
  [rx_crc_err1] -> rst_delay4/1
  [cnt_rst] -> Subsystem9/1(rst)
  [ct_bank_error_g0] -> Subsystem9/2(in0)
  [cnt_rst] -> Subsystem22/1(rst)
  rst_delay7/1 -> status0/3(out_hmc_post_pol1)
  rst_delay5/1 -> status0/4(out_hmc_init_pol1)
  rst_delay2/1 -> status0/1(out_hmc_post_pol0)
  rst_delay1/1 -> status0/2(out_hmc_init_pol0)
  [postokay0] -> rst_delay2/1
  [init_done0] -> rst_delay1/1
  [init_done1] -> rst_delay5/1
  [postokay1] -> rst_delay7/1
  [ct_bank_error_g1] -> Subsystem9/3(in1)
  [obuf_ct_addr_err_g] -> Subsystem9/4(in2)
  [rd_go_err_g] -> Subsystem9/5(in3)
  Subsystem9/1(out0) -> status3/1(out_bank_err_cnt_pol0)
  Subsystem9/2(out1) -> status3/2(out_bank_err_cnt_pol1)
  Subsystem9/3(out2) -> status3/3(out_obuff_bank_err_cnt)
  Subsystem9/4(out3) -> status3/4(out_rd_go_err_cnt)
  rst_delay3/1 -> status1/1(out_hmc_crc_err_cnt_pol0)
  rst_delay4/1 -> status1/2(out_hmc_crc_err_cnt_pol1)
  Subsystem22/1(out0) -> status4/1(out_sync_in_err_cnt)
  Subsystem22/2(out1) -> status4/2(out_fifo_full_err_cnt)
  Subsystem22/3(out2) -> status4/3(out_reorder_missing_err_cnt)
  [cthmc_sync_err_g0] -> Subsystem22/2(in0)
  [hmc_fifo_full_g] -> Subsystem22/3(in1)
  [obuf_proc_err_miss_0_g] -> Subsystem22/4(in2)
  [hmc_wr_rdy_0] -> Inverter1/1
  [hmc_rd_rdy_0] -> Inverter2/1
  [hmc_wr_rdy_1] -> Inverter22/1
  [hmc_rd_rdy_1] -> Inverter23/1
  Inverter2/1 -> Logical4/5
  Inverter1/1 -> Logical4/4
  Inverter22/1 -> Logical4/2
  [hmc_fifo_full_g] -> Delay19/1
  Inverter23/1 -> Logical4/3
  Logical4/1 -> error0/1
  [cnt_rst] -> Subsystem/1(In1)
  [hmc_rd_rdy_0] -> Subsystem/2(In2)
  [hmc_wr_rdy_0] -> Subsystem/3(In3)
  [hmc_rd_rdy_1] -> Subsystem/4(In4)
  [hmc_wr_rdy_1] -> Subsystem/5(In5)
  Subsystem/1(Out1) -> status2/1(out_hmc_overflow_err_cnt_pol0)
  Subsystem/2(Out2) -> status2/2(out_hmc_overflow_err_cnt_pol1)
  Delay19/1 -> Logical4/1
  [ct_tvg_en] -> Mux4/1
  tvg_data_tone_gen/1(d) -> Mux4/4
  Delay41/1 -> Mux4/2
  in_d1/1 -> Delay41/1
  Delay46/1 -> Concat3/3, Delay47/1
  Delay47/1 -> Concat3/2, Delay51/1
  Delay51/1 -> Concat3/1
  Constant12/1 -> Relational/2
  Counter/1 -> Gateway Out2/1, Relational/1
  Relational/1 -> Logical1/1
  Gateway Out/1 -> Scope/1
  Gateway Out1/1 -> Scope/2
  Gateway Out2/1 -> Scope/3
  Gateway Out3/1 -> Scope/4
  Concat2/1 -> Delay78/1
  Mux4/1 -> Concat2/4, Delay60/1  "data128"
  Delay60/1 -> Delay64/1, Concat2/3
  Delay64/1 -> Delay65/1, Concat2/2
  Delay65/1 -> Concat2/1
  Delay75/1 -> [d256_1]
  Delay78/1 -> Delay75/1, Delay81/1
  [dv256] -> hmc_addr_gen/2(dv)
  [d256_1] -> hmc_addr_gen/4(d256_1)
  hmc_addr_gen/2(wr_en) -> [wr_en]
  hmc_addr_gen/3(wr_addr) -> [wr_addr]
  hmc_addr_gen/4(wr_d256_0) -> [wr_d256_0]
  hmc_addr_gen/5(wr_d256_1) -> [wr_d256_1]
  hmc_addr_gen/6(rd_en) -> [rd_en]
  hmc_addr_gen/8(rd_tag) -> [rd_tag]
  hmc_addr_gen/7(rd_addr) -> [rd_addr]
  hmc_addr_gen/9(rd_addr_arm) -> [rd_addr_arm]
  [rd_en] -> [rd_en_0]
  tvg_data_gen1/1(d) -> Mux4/3
  tvg_time_ramp_gen0/1(d) -> Mux3/3
  tvg_freq_ramp_gen0/1(d) -> Mux3/5
  tvg_freq_ramp_gen1/1(d) -> Mux4/5
  Gateway Out8/1 -> Scope2/1
  Gateway Out9/1 -> Scope2/2
  Gateway Out10/1 -> Scope2/3
  Gateway Out11/1 -> Scope2/4
  Delay39/1 -> Gateway Out1/1, Counter/2, Delay54/1, Delay60/2, Delay64/2, Delay65/2, Delay46/2, Delay47/2, Delay51/2, Logical1/2
  Delay54/1 -> Delay83/1, Delay79/1
  Slice/1 -> Gateway Out11/1
  [tvgtone_p0] -> tvg_data_tone_gen1/3(target)
  [tvgtone_level0] -> tvg_data_tone_gen1/4(level)
  tvg_data_tone_gen1/1(d) -> Mux3/4
  Logical1/1 -> Delay1/1, Gateway Out3/1
  Delay14/1 -> Slice/1
  Delay77/1 -> Gateway Out10/1
  Delay79/1 -> Gateway Out9/1
  Delay80/1 -> Gateway Out8/1
  Gateway Out6/1 -> Scope1/1
  Gateway Out7/1 -> Scope1/2
  Gateway Out4/1 -> Scope1/3
  Gateway Out5/1 -> Scope1/4
  Slice1/1 -> Gateway Out5/1
  Delay81/1 -> Slice1/1
  Delay82/1 -> Gateway Out4/1
  Delay83/1 -> Gateway Out7/1
  Delay84/1 -> Gateway Out6/1
  [wr_sync] -> [wr_sync_0]
  [wr_en] -> [wr_en_0]
  [wr_en] -> [wr_en_1]
  [wr_addr] -> [wr_addr_1]
  [rd_en] -> [rd_en_1]
  [rd_addr] -> [rd_addr_0]
  [rd_tag] -> [rd_tag_1]
  Delay4/1 -> [hmc_d256_1]
  [hmc_d256_1_tmp] -> Delay4/1
  [hmc_tag_1_tmp] -> Delay17/1
  Delay17/1 -> [hmc_tag_1]
  [hmc_dv_1_tmp] -> Delay18/1
  Delay18/1 -> [hmc_dv_1]
  Constant13/1 -> [hmc_fifo_full_g]
  [hmc_d256_0] -> Delay9/1
  [obuf_proc_err_miss_1_g] -> Subsystem22/5(in3)
  Subsystem22/4(out3) -> status4/4(out_reorder_missing_err_cnt1)
  [hmc_dv_1] -> Delay11/1
  Delay11/1 -> obuf/5(dv1)
  [hmc_tag_1] -> Delay12/1
  Delay12/1 -> obuf/6(tag1)
  Delay13/1 -> obuf/7(din1)
  [hmc_d256_1] -> Delay13/1
  [ct_tvg_en] -> Subsystem1/3(tvg_sel)
  Delay25/1 -> Delay63/1
  Delay26/1 -> Delay48/1, Delay21/2, Delay22/2, Delay66/1
  Delay27/1 -> Delay22/1, Relational1/2, Delay72/1
  Delay28/1 -> Delay73/1
  Delay29/1 -> Delay85/1
  Delay40/1 -> Delay86/1
  Delay61/1 -> Delay94/1
  Delay62/1 -> Delay95/1
  Subsystem1/1(dout) -> Relational1/1, Delay21/1
  Delay63/1 -> out_sync/1, Gateway Out12/1, Gateway Out20/1
  Delay66/1 -> out_dv/1, Gateway Out13/1, Gateway Out21/1
  Delay72/1 -> out_d256/1
  Delay73/1 -> pkt_start/1, Gateway Out14/1, Gateway Out22/1
  Delay85/1 -> [raw_freq_ctr_g]
  Delay86/1 -> freq_id/1, Gateway Out15/1
  Delay94/1 -> x_index/1, Gateway Out23/1
  Delay95/1 -> x_pkt_index/1
  Relational1/1 -> tvg_error/1
  Delay/1 -> Subsystem1/1(rst), Delay25/1
  Gateway Out12/1 -> Scope3/1
  Gateway Out13/1 -> Scope3/2
  Gateway Out14/1 -> Scope3/3
  Gateway Out15/1 -> Scope3/4
  Gateway Out20/1 -> Scope5/1
  Gateway Out21/1 -> Scope5/2
  Gateway Out22/1 -> Scope5/3
  Gateway Out23/1 -> Scope5/4
  Gateway Out33/1 -> Scope9/1
  Gateway Out34/1 -> Scope9/2
  Gateway Out35/1 -> Scope9/3
  Gateway Out36/1 -> Scope9/4
  Gateway Out41/1 -> Scope11/1
  Gateway Out42/1 -> Scope11/2
  Gateway Out43/1 -> Scope11/3
  Gateway Out44/1 -> Scope11/4
  Gateway Out45/1 -> Scope13/1
  Gateway Out46/1 -> Scope13/2
  Gateway Out47/1 -> Scope13/3
  Gateway Out48/1 -> Scope13/4
  Gateway Out49/1 -> Scope12/1
  Gateway Out50/1 -> Scope12/2
  Gateway Out51/1 -> Scope12/3
  Gateway Out52/1 -> Scope12/4
  Gateway Out37/1 -> Scope16/1
  Gateway Out38/1 -> Scope16/2
  Gateway Out39/1 -> Scope16/3
  Gateway Out40/1 -> Scope16/4
  Gateway Out53/1 -> Scope10/1
  Gateway Out54/1 -> Scope10/2
  Gateway Out55/1 -> Scope10/3
  Gateway Out56/1 -> Scope10/4
  Gateway Out57/1 -> Scope15/1
  Gateway Out58/1 -> Scope15/2
  Gateway Out59/1 -> Scope15/3
  Gateway Out60/1 -> Scope15/4
  Gateway Out61/1 -> Scope14/1
  Gateway Out62/1 -> Scope14/2
  Gateway Out63/1 -> Scope14/3
  Gateway Out64/1 -> Scope14/4
  bus_expand/1(msb_out16) -> Gateway Out35/1, Relational6/1
  bus_expand1/1(msb_out16) -> Gateway Out36/1, Relational6/2
  Relational6/1 -> Gateway Out34/1
  Relational7/1 -> Gateway Out42/1
  bus_expand/2(out15) -> Gateway Out43/1, Relational7/1
  bus_expand1/2(out15) -> Gateway Out44/1, Relational7/2
  bus_expand1/3(out14) -> Relational8/2, Gateway Out48/1
  bus_expand/3(out14) -> Gateway Out47/1, Relational8/1
  Relational8/1 -> Gateway Out46/1
  Relational9/1 -> Gateway Out50/1
  bus_expand/4(out13) -> Gateway Out51/1, Relational9/1
  bus_expand1/4(out13) -> Gateway Out52/1, Relational9/2
  Relational10/1 -> Gateway Out38/1
  bus_expand/5(out12) -> Gateway Out39/1, Relational10/1
  bus_expand1/5(out12) -> Relational10/2, Gateway Out40/1
  Relational11/1 -> Gateway Out54/1
  bus_expand/6(out11) -> Gateway Out55/1, Relational11/1
  bus_expand1/6(out11) -> Relational11/2, Gateway Out56/1
  Relational12/1 -> Gateway Out58/1
  bus_expand/7(out10) -> Gateway Out59/1, Relational12/1
  bus_expand1/7(out10) -> Gateway Out60/1, Relational12/2
  Relational13/1 -> Gateway Out62/1
  bus_expand/8(out9) -> Gateway Out63/1, Relational13/1
  Gateway Out73/1 -> Scope20/1
  Gateway Out74/1 -> Scope20/2
  Gateway Out75/1 -> Scope20/3
  Gateway Out76/1 -> Scope20/4
  Relational14/1 -> Gateway Out74/1, Gateway Out16/1
  bus_expand1/16(lsb_out1) -> Gateway Out19/1, Relational18/1, Gateway Out76/1, Relational14/2
  bus_expand/16(lsb_out1) -> Delay23/1, Gateway Out75/1, Relational14/1
  Delay21/1 -> bus_expand/1(bus_in)
  Delay22/1 -> bus_expand1/1(bus_in)
  Gateway Out24/1 -> Scope6/1
  Gateway Out25/1 -> Scope6/2
  Gateway Out26/1 -> Scope6/3
  Gateway Out27/1 -> Scope6/4
  Relational2/1 -> Gateway Out25/1
  Delay48/1 -> Gateway Out28/1, Gateway Out32/1, Gateway Out68/1, Gateway Out72/1, Gateway Out80/1, Gateway Out84/1, Delay23/2, Gateway Out17/1, Counter1/2, Gateway Out73/1, Gateway Out24/1, Gateway Out61/1, Gateway Out57/1, Gateway Out53/1, Gateway Out37/1, Gateway Out49/1, Gateway Out45/1, Gateway Out41/1, Gateway Out33/1
  bus_expand/9(out8) -> Gateway Out26/1, Relational2/1
  bus_expand1/9(out8) -> Gateway Out27/1, Relational2/2
  Gateway Out28/1 -> Scope7/1
  Gateway Out29/1 -> Scope7/2
  Gateway Out30/1 -> Scope7/3
  Gateway Out31/1 -> Scope7/4
  Relational3/1 -> Gateway Out29/1
  bus_expand/10(out7) -> Gateway Out30/1, Relational3/1
  bus_expand1/10(out7) -> Gateway Out31/1, Relational3/2
  Gateway Out32/1 -> Scope8/1
  Gateway Out65/1 -> Scope8/2
  Gateway Out66/1 -> Scope8/3
  Gateway Out67/1 -> Scope8/4
  Relational4/1 -> Gateway Out65/1
  bus_expand1/8(out9) -> Gateway Out64/1, Relational13/2
  bus_expand1/11(out6) -> Gateway Out67/1, Relational4/2
  bus_expand/11(out6) -> Gateway Out66/1, Relational4/1
  Gateway Out68/1 -> Scope17/1
  Gateway Out69/1 -> Scope17/2
  Gateway Out70/1 -> Scope17/3
  Gateway Out71/1 -> Scope17/4
  Gateway Out72/1 -> Scope4/1
  Gateway Out77/1 -> Scope4/2
  Gateway Out78/1 -> Scope4/3
  Gateway Out79/1 -> Scope4/4
  Relational5/1 -> Gateway Out69/1
  bus_expand/12(out5) -> Gateway Out70/1, Relational5/1
  bus_expand1/12(out5) -> Gateway Out71/1, Relational5/2
  Relational15/1 -> Gateway Out77/1
  bus_expand/13(out4) -> Gateway Out78/1, Relational15/1
  bus_expand1/13(out4) -> Gateway Out79/1, Relational15/2
  Gateway Out80/1 -> Scope18/1
  Gateway Out81/1 -> Scope18/2
  Gateway Out82/1 -> Scope18/3
  Gateway Out83/1 -> Scope18/4
  Relational16/1 -> Gateway Out81/1
  bus_expand/14(out3) -> Gateway Out82/1, Relational16/1
  bus_expand1/14(out3) -> Gateway Out83/1, Relational16/2
  Gateway Out84/1 -> Scope19/1
  Gateway Out85/1 -> Scope19/2
  Gateway Out86/1 -> Scope19/3
  Gateway Out87/1 -> Scope19/4
  Relational17/1 -> Gateway Out85/1
  bus_expand/15(out2) -> Gateway Out86/1, Relational17/1
  bus_expand1/15(out2) -> Gateway Out87/1, Relational17/2
  Gateway Out16/1 -> Scope21/1
  Gateway Out17/1 -> Scope21/2
  Gateway Out18/1 -> Scope21/3
  Gateway Out19/1 -> Scope21/4
  Relational18/1 -> Counter1/1
  Delay23/1 -> Relational18/2
  Counter1/1 -> Gateway Out18/1
  pipeline4/1(q) -> [hmc_d256_0_tmp]
  Constant9/1 -> hmc1/10
  hmc/10 -> Terminator5/1
  [wr_en_1] -> Logical18/2  "WR_en"
  hmc/9 -> Terminator4/1
  hmc1/2 -> convert_rd_en1/1
  hmc1/1 -> pipeline7/1(d)  "hmc_d256"
  hmc1/7 -> Terminator11/1
  [rd_tag_1] -> pipeline13/1(d)  "RD_tag"
  hmc/6 -> Terminator1/1
  pipeline10/1(q) -> hmc1/2, [wr_addr_final_g1]
  Constant14/1 -> [errstat0]
  [rd_en_1] -> Logical2/2  "RD_en"
  pipeline7/1(q) -> [hmc_d256_1_tmp]
  hmc/4 -> [hmc_rd_rdy_0]
  pipeline3/1(q) -> hmc/6, [rd_tag_final_g0]
  [init_done0] -> Logical7/1
  pipeline1/1(q) -> hmc/3, [wr_data_final_g0]
  hmc1/8 -> Terminator12/1
  [rd_tag_0] -> pipeline3/1(d)  "RD_tag"
  Constant6/1 -> hmc1/7
  hmc1/9 -> Terminator13/1
  hmc1/5 -> pipeline9/1(d)
  Logical11/1 -> hmc/4, [rd_en_final_g0]
  Constant16/1 -> [errstat1]
  [postokay0] -> Logical7/2
  Constant/1 -> hmc/7
  Constant17/1 -> [rx_crc_err1]
  [wr_addr_1] -> pipeline10/1(d)  "WR_addr"
  Logical28/1 -> Logical2/1, Logical18/1
  Constant8/1 -> hmc1/9
  pipeline8/1(q) -> [hmc_dv_1_tmp]  "hmc_dv"
  pipeline2/1(q) -> hmc/5, [rd_addr_final_g0]
  hmc/1 -> pipeline4/1(d)  "hmc_d256"
  hmc/7 -> Terminator2/1
  [init_done1] -> Logical28/1
  Constant4/1 -> hmc/11
  hmc1/6 -> Terminator10/1
  [wr_addr_0] -> pipeline/1(d)  "WR_addr"
  [wr_en_0] -> Logical5/2  "WR_en"
  Constant1/1 -> hmc/8
  hmc/2 -> convert_rd_en4/1
  [wr_d256_0] -> pipeline1/1(d)
  hmc1/3 -> [hmc_wr_rdy_1]
  pipeline11/1(q) -> [wr_data_final_g1], hmc1/3
  Logical5/1 -> hmc/1, [wr_en_final_g0]
  Constant7/1 -> hmc1/8
  [rd_addr_0] -> pipeline2/1(d)  "RD_rdaddr"
  Logical18/1 -> [wr_en_final_g1], hmc1/1
  pipeline/1(q) -> [wr_addr_final_g0], hmc/2
  pipeline12/1(q) -> [rd_addr_final_g1], hmc1/5
  hmc/3 -> [hmc_wr_rdy_0]
  [wr_d256_1] -> pipeline11/1(d)
  Constant3/1 -> hmc/10
  Logical2/1 -> [rd_en_final_g1], hmc1/4
  pipeline9/1(q) -> [hmc_tag_1_tmp]  "hmc_tag"
  [postokay1] -> Logical28/2
  hmc/5 -> pipeline6/1(d)
  hmc1/11 -> [postokay1], [init_done1]
  pipeline6/1(q) -> [hmc_tag_0_tmp]  "hmc_tag"
  pipeline5/1(q) -> [hmc_dv_0_tmp]  "hmc_dv"
  hmc/11 -> [postokay0], [init_done0]
  Logical7/1 -> Logical11/1, Logical5/1
  hmc1/10 -> Terminator14/1
  [rd_en_0] -> Logical11/2  "RD_en"
  [rd_addr_1] -> pipeline12/1(d)  "RD_rdaddr"
  Constant5/1 -> hmc/12
  Constant11/1 -> hmc1/12
  pipeline13/1(q) -> hmc1/6
  convert_rd_en1/1 -> pipeline8/1(d)  "hmcout_dv"
  hmc/8 -> Terminator3/1
  hmc1/4 -> [hmc_rd_rdy_1]
  Constant2/1 -> hmc/9
  [rd_addr_arm] -> edge_detect1/1(in)
  convert_rd_en4/1 -> pipeline5/1(d)  "hmcout_dv"
  Constant10/1 -> hmc1/11
  Constant15/1 -> [rx_crc_err0]
  edge_detect1/1(out) -> [hmc_sync_tmp]
